simulink model "PI_D_controller"  (R2024b)
settings: Solver=VariableStepAuto  StartTime=0.0  StopTime=10.0  RelTol=1e-3
settings Model: Creator=emrekarausta  LastModifiedBy=emrekarausta

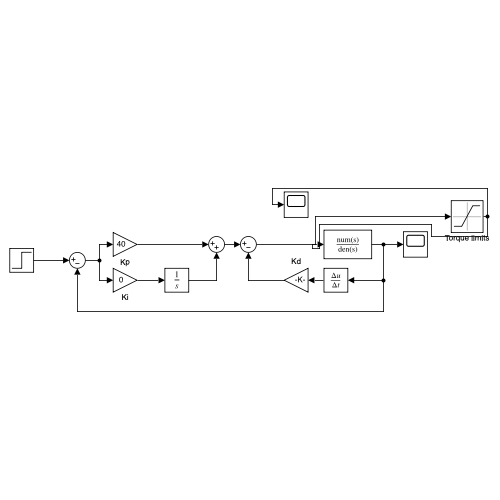
[thumbnail: Simulink's stored preview of the top-level diagram]
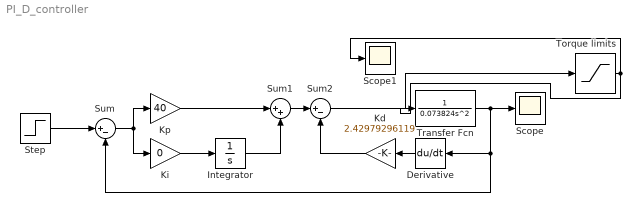
== system PI_D_controller ==
  Derivative : Derivative
  Integrator : Integrator
  Kd : Gain  Gain=2.42979296119
  Ki : Gain  Gain=0
  Kp : Gain  Gain=40
  Scope : Scope
  Scope1 : Scope
  Step : Step  Time=0  After=0.25  SampleTime=0
  Sum : Sum  Inputs=|+-
  Sum1 : Sum  Inputs=|++
  Sum2 : Sum  Inputs=|+-
  Torque limits : Saturate  UpperLimit=10  LowerLimit=-6
  Transfer Fcn : TransferFcn  Denominator=[0.073824 0 0]
  wires:
  Sum1/1 -> Sum2/1
  Derivative/1 -> Kd/1
  Transfer Fcn/1 -> Derivative/1, Sum/2, Scope/1
  Kd/1 -> Sum2/2
  Step/1 -> Sum/1
  Sum/1 -> Ki/1, Kp/1
  Ki/1 -> Integrator/1
  Integrator/1 -> Sum1/2
  Kp/1 -> Sum1/1
  Sum2/1 -> Torque limits/1
  Torque limits/1 -> Transfer Fcn/1, Scope1/1
